simulink model "IEEE33_TR_TEMPORAL_RECOGNIZABILITY_MASTER"  (R2026b)
settings: Solver=ode23t  StopTime=0.2  MaxStep=1e-5
undefined symbols (not defined in the file): Three_PhaseBreaker_class, Three_PhaseSeriesRLCLoad_class, Three_PhaseSource_class, Three_PhaseV_IMeasuremen_class
libraries: ee_lib x146, nesl_utility x106, fl_lib x33, eeRmsMeasurement x2
(part 3 of 7)

== system IEEE33_TR_TEMPORAL_RECOGNIZABILITY_MASTER/Three-Phase Series RLC Branch31 ==
  Three_PhaseSeriesRLCBran : ee_lib/Passive/RLC Assemblies/RLC (Three-Phase)  port_option=ee.enum.threePhasePort.expanded  component_structure=4  R=0.5075 Ohm  L=0.00082283 H  C=1e-06 F  R_parasitic=1e-6 Ohm  G_parasitic=1e-6 1/Ohm  IL_specify=on  IL_priority=High  IL=[0, 0, 0] A  IL_nominal_specify=off  IL_nominal_value=1  IL_nominal_unit=A  VC_specify=on  VC_priority=High  VC=[0, 0, 0] V  VC_nominal_specify=off  VC_nominal_value=1  VC_nominal_unit=V
  A : PMIOPort  Side=Left
  B : PMIOPort  Port=2  Side=Left
  C : PMIOPort  Port=3  Side=Left
  a : PMIOPort  Port=4  Side=Right
  b : PMIOPort  Port=5  Side=Right
  c : PMIOPort  Port=6  Side=Right
  connections:
  Three_PhaseSeriesRLCBran/RConn3 -- c/RConn1
  Three_PhaseSeriesRLCBran/RConn2 -- b/RConn1
  Three_PhaseSeriesRLCBran/RConn1 -- a/RConn1
  C/RConn1 -- Three_PhaseSeriesRLCBran/LConn3
  B/RConn1 -- Three_PhaseSeriesRLCBran/LConn2
  A/RConn1 -- Three_PhaseSeriesRLCBran/LConn1

== system IEEE33_TR_TEMPORAL_RECOGNIZABILITY_MASTER/Three-Phase Series RLC Branch32 ==
  Three_PhaseSeriesRLCBran : ee_lib/Passive/RLC Assemblies/RLC (Three-Phase)  port_option=ee.enum.threePhasePort.expanded  component_structure=4  R=0.9744 Ohm  L=0.0030653 H  C=1e-06 F  R_parasitic=1e-6 Ohm  G_parasitic=1e-6 1/Ohm  IL_specify=on  IL_priority=High  IL=[0, 0, 0] A  IL_nominal_specify=off  IL_nominal_value=1  IL_nominal_unit=A  VC_specify=on  VC_priority=High  VC=[0, 0, 0] V  VC_nominal_specify=off  VC_nominal_value=1  VC_nominal_unit=V
  A : PMIOPort  Side=Left
  B : PMIOPort  Port=2  Side=Left
  C : PMIOPort  Port=3  Side=Left
  a : PMIOPort  Port=4  Side=Right
  b : PMIOPort  Port=5  Side=Right
  c : PMIOPort  Port=6  Side=Right
  connections:
  Three_PhaseSeriesRLCBran/RConn3 -- c/RConn1
  Three_PhaseSeriesRLCBran/RConn2 -- b/RConn1
  Three_PhaseSeriesRLCBran/RConn1 -- a/RConn1
  C/RConn1 -- Three_PhaseSeriesRLCBran/LConn3
  B/RConn1 -- Three_PhaseSeriesRLCBran/LConn2
  A/RConn1 -- Three_PhaseSeriesRLCBran/LConn1

== system IEEE33_TR_TEMPORAL_RECOGNIZABILITY_MASTER/Three-Phase Series RLC Branch33 ==
  Three_PhaseSeriesRLCBran : ee_lib/Passive/RLC Assemblies/RLC (Three-Phase)  port_option=ee.enum.threePhasePort.expanded  component_structure=4  R=0.3105 Ohm  L=0.001152 H  C=1e-06 F  R_parasitic=1e-6 Ohm  G_parasitic=1e-6 1/Ohm  IL_specify=on  IL_priority=High  IL=[0, 0, 0] A  IL_nominal_specify=off  IL_nominal_value=1  IL_nominal_unit=A  VC_specify=on  VC_priority=High  VC=[0, 0, 0] V  VC_nominal_specify=off  VC_nominal_value=1  VC_nominal_unit=V
  A : PMIOPort  Side=Left
  B : PMIOPort  Port=2  Side=Left
  C : PMIOPort  Port=3  Side=Left
  a : PMIOPort  Port=4  Side=Right
  b : PMIOPort  Port=5  Side=Right
  c : PMIOPort  Port=6  Side=Right
  connections:
  Three_PhaseSeriesRLCBran/RConn3 -- c/RConn1
  Three_PhaseSeriesRLCBran/RConn2 -- b/RConn1
  Three_PhaseSeriesRLCBran/RConn1 -- a/RConn1
  C/RConn1 -- Three_PhaseSeriesRLCBran/LConn3
  B/RConn1 -- Three_PhaseSeriesRLCBran/LConn2
  A/RConn1 -- Three_PhaseSeriesRLCBran/LConn1

== system IEEE33_TR_TEMPORAL_RECOGNIZABILITY_MASTER/Three-Phase Series RLC Branch34 ==
  Three_PhaseSeriesRLCBran : ee_lib/Passive/RLC Assemblies/RLC (Three-Phase)  port_option=ee.enum.threePhasePort.expanded  component_structure=4  R=0.341 Ohm  L=0.0016877 H  C=1e-06 F  R_parasitic=1e-6 Ohm  G_parasitic=1e-6 1/Ohm  IL_specify=on  IL_priority=High  IL=[0, 0, 0] A  IL_nominal_specify=off  IL_nominal_value=1  IL_nominal_unit=A  VC_specify=on  VC_priority=High  VC=[0, 0, 0] V  VC_nominal_specify=off  VC_nominal_value=1  VC_nominal_unit=V
  A : PMIOPort  Side=Left
  B : PMIOPort  Port=2  Side=Left
  C : PMIOPort  Port=3  Side=Left
  a : PMIOPort  Port=4  Side=Right
  b : PMIOPort  Port=5  Side=Right
  c : PMIOPort  Port=6  Side=Right
  connections:
  Three_PhaseSeriesRLCBran/RConn3 -- c/RConn1
  Three_PhaseSeriesRLCBran/RConn2 -- b/RConn1
  Three_PhaseSeriesRLCBran/RConn1 -- a/RConn1
  C/RConn1 -- Three_PhaseSeriesRLCBran/LConn3
  B/RConn1 -- Three_PhaseSeriesRLCBran/LConn2
  A/RConn1 -- Three_PhaseSeriesRLCBran/LConn1

== system IEEE33_TR_TEMPORAL_RECOGNIZABILITY_MASTER/Three-Phase Series RLC Branch35 ==
  Three_PhaseSeriesRLCBran : ee_lib/Passive/RLC Assemblies/RLC (Three-Phase)  port_option=ee.enum.threePhasePort.expanded  component_structure=4  R=2 Ohm  L=0.0063662 H  C=1e-06 F  R_parasitic=1e-6 Ohm  G_parasitic=1e-6 1/Ohm  IL_specify=on  IL_priority=High  IL=[0, 0, 0] A  IL_nominal_specify=off  IL_nominal_value=1  IL_nominal_unit=A  VC_specify=on  VC_priority=High  VC=[0, 0, 0] V  VC_nominal_specify=off  VC_nominal_value=1  VC_nominal_unit=V
  A : PMIOPort  Side=Left
  B : PMIOPort  Port=2  Side=Left
  C : PMIOPort  Port=3  Side=Left
  a : PMIOPort  Port=4  Side=Right
  b : PMIOPort  Port=5  Side=Right
  c : PMIOPort  Port=6  Side=Right
  connections:
  Three_PhaseSeriesRLCBran/RConn3 -- c/RConn1
  Three_PhaseSeriesRLCBran/RConn2 -- b/RConn1
  Three_PhaseSeriesRLCBran/RConn1 -- a/RConn1
  C/RConn1 -- Three_PhaseSeriesRLCBran/LConn3
  B/RConn1 -- Three_PhaseSeriesRLCBran/LConn2
  A/RConn1 -- Three_PhaseSeriesRLCBran/LConn1

== system IEEE33_TR_TEMPORAL_RECOGNIZABILITY_MASTER/Three-Phase Series RLC Branch36 ==
  Three_PhaseSeriesRLCBran : ee_lib/Passive/RLC Assemblies/RLC (Three-Phase)  port_option=ee.enum.threePhasePort.expanded  component_structure=4  R=2 Ohm  L=0.0063662 H  C=1e-06 F  R_parasitic=1e-6 Ohm  G_parasitic=1e-6 1/Ohm  IL_specify=on  IL_priority=High  IL=[0, 0, 0] A  IL_nominal_specify=off  IL_nominal_value=1  IL_nominal_unit=A  VC_specify=on  VC_priority=High  VC=[0, 0, 0] V  VC_nominal_specify=off  VC_nominal_value=1  VC_nominal_unit=V
  A : PMIOPort  Side=Left
  B : PMIOPort  Port=2  Side=Left
  C : PMIOPort  Port=3  Side=Left
  a : PMIOPort  Port=4  Side=Right
  b : PMIOPort  Port=5  Side=Right
  c : PMIOPort  Port=6  Side=Right
  connections:
  Three_PhaseSeriesRLCBran/RConn3 -- c/RConn1
  Three_PhaseSeriesRLCBran/RConn2 -- b/RConn1
  Three_PhaseSeriesRLCBran/RConn1 -- a/RConn1
  C/RConn1 -- Three_PhaseSeriesRLCBran/LConn3
  B/RConn1 -- Three_PhaseSeriesRLCBran/LConn2
  A/RConn1 -- Three_PhaseSeriesRLCBran/LConn1

== system IEEE33_TR_TEMPORAL_RECOGNIZABILITY_MASTER/Three-Phase Series RLC Branch37 ==
  Three_PhaseSeriesRLCBran : ee_lib/Passive/RLC Assemblies/RLC (Three-Phase)  port_option=ee.enum.threePhasePort.expanded  component_structure=4  R=0.5 Ohm  L=0.0015915 H  C=1e-06 F  R_parasitic=1e-6 Ohm  G_parasitic=1e-6 1/Ohm  IL_specify=on  IL_priority=High  IL=[0, 0, 0] A  IL_nominal_specify=off  IL_nominal_value=1  IL_nominal_unit=A  VC_specify=on  VC_priority=High  VC=[0, 0, 0] V  VC_nominal_specify=off  VC_nominal_value=1  VC_nominal_unit=V
  A : PMIOPort  Side=Left
  B : PMIOPort  Port=2  Side=Left
  C : PMIOPort  Port=3  Side=Left
  a : PMIOPort  Port=4  Side=Right
  b : PMIOPort  Port=5  Side=Right
  c : PMIOPort  Port=6  Side=Right
  connections:
  Three_PhaseSeriesRLCBran/RConn3 -- c/RConn1
  Three_PhaseSeriesRLCBran/RConn2 -- b/RConn1
  Three_PhaseSeriesRLCBran/RConn1 -- a/RConn1
  C/RConn1 -- Three_PhaseSeriesRLCBran/LConn3
  B/RConn1 -- Three_PhaseSeriesRLCBran/LConn2
  A/RConn1 -- Three_PhaseSeriesRLCBran/LConn1

== system IEEE33_TR_TEMPORAL_RECOGNIZABILITY_MASTER/Three-Phase Series RLC Branch38 ==
  Three_PhaseSeriesRLCBran : ee_lib/Passive/RLC Assemblies/RLC (Three-Phase)  port_option=ee.enum.threePhasePort.expanded  component_structure=4  R=0.5 Ohm  L=0.0015915 H  C=1e-06 F  R_parasitic=1e-6 Ohm  G_parasitic=1e-6 1/Ohm  IL_specify=on  IL_priority=High  IL=[0, 0, 0] A  IL_nominal_specify=off  IL_nominal_value=1  IL_nominal_unit=A  VC_specify=on  VC_priority=High  VC=[0, 0, 0] V  VC_nominal_specify=off  VC_nominal_value=1  VC_nominal_unit=V
  A : PMIOPort  Side=Left
  B : PMIOPort  Port=2  Side=Left
  C : PMIOPort  Port=3  Side=Left
  a : PMIOPort  Port=4  Side=Right
  b : PMIOPort  Port=5  Side=Right
  c : PMIOPort  Port=6  Side=Right
  connections:
  Three_PhaseSeriesRLCBran/RConn3 -- c/RConn1
  Three_PhaseSeriesRLCBran/RConn2 -- b/RConn1
  Three_PhaseSeriesRLCBran/RConn1 -- a/RConn1
  C/RConn1 -- Three_PhaseSeriesRLCBran/LConn3
  B/RConn1 -- Three_PhaseSeriesRLCBran/LConn2
  A/RConn1 -- Three_PhaseSeriesRLCBran/LConn1

== system IEEE33_TR_TEMPORAL_RECOGNIZABILITY_MASTER/Three-Phase Series RLC Branch4 ==
  Three_PhaseSeriesRLCBran : ee_lib/Passive/RLC Assemblies/RLC (Three-Phase)  port_option=ee.enum.threePhasePort.expanded  component_structure=4  R=0.819 Ohm  L=0.0022505 H  C=1e-06 F  R_parasitic=1e-6 Ohm  G_parasitic=1e-6 1/Ohm  IL_specify=on  IL_priority=High  IL=[0, 0, 0] A  IL_nominal_specify=off  IL_nominal_value=1  IL_nominal_unit=A  VC_specify=on  VC_priority=High  VC=[0, 0, 0] V  VC_nominal_specify=off  VC_nominal_value=1  VC_nominal_unit=V
  A : PMIOPort  Side=Left
  B : PMIOPort  Port=2  Side=Left
  C : PMIOPort  Port=3  Side=Left
  a : PMIOPort  Port=4  Side=Right
  b : PMIOPort  Port=5  Side=Right
  c : PMIOPort  Port=6  Side=Right
  connections:
  Three_PhaseSeriesRLCBran/RConn3 -- c/RConn1
  Three_PhaseSeriesRLCBran/RConn2 -- b/RConn1
  Three_PhaseSeriesRLCBran/RConn1 -- a/RConn1
  C/RConn1 -- Three_PhaseSeriesRLCBran/LConn3
  B/RConn1 -- Three_PhaseSeriesRLCBran/LConn2
  A/RConn1 -- Three_PhaseSeriesRLCBran/LConn1

== system IEEE33_TR_TEMPORAL_RECOGNIZABILITY_MASTER/Three-Phase Series RLC Branch5 ==
  Three_PhaseSeriesRLCBran : ee_lib/Passive/RLC Assemblies/RLC (Three-Phase)  port_option=ee.enum.threePhasePort.expanded  component_structure=4  R=0.1872 Ohm  L=0.0019697 H  C=1e-06 F  R_parasitic=1e-6 Ohm  G_parasitic=1e-6 1/Ohm  IL_specify=on  IL_priority=High  IL=[0, 0, 0] A  IL_nominal_specify=off  IL_nominal_value=1  IL_nominal_unit=A  VC_specify=on  VC_priority=High  VC=[0, 0, 0] V  VC_nominal_specify=off  VC_nominal_value=1  VC_nominal_unit=V
  A : PMIOPort  Side=Left
  B : PMIOPort  Port=2  Side=Left
  C : PMIOPort  Port=3  Side=Left
  a : PMIOPort  Port=4  Side=Right
  b : PMIOPort  Port=5  Side=Right
  c : PMIOPort  Port=6  Side=Right
  connections:
  Three_PhaseSeriesRLCBran/RConn3 -- c/RConn1
  Three_PhaseSeriesRLCBran/RConn2 -- b/RConn1
  Three_PhaseSeriesRLCBran/RConn1 -- a/RConn1
  C/RConn1 -- Three_PhaseSeriesRLCBran/LConn3
  B/RConn1 -- Three_PhaseSeriesRLCBran/LConn2
  A/RConn1 -- Three_PhaseSeriesRLCBran/LConn1

== system IEEE33_TR_TEMPORAL_RECOGNIZABILITY_MASTER/Three-Phase Series RLC Branch6 ==
  Three_PhaseSeriesRLCBran : ee_lib/Passive/RLC Assemblies/RLC (Three-Phase)  port_option=ee.enum.threePhasePort.expanded  component_structure=4  R=0.7114 Ohm  L=0.00074835 H  C=1e-06 F  R_parasitic=1e-6 Ohm  G_parasitic=1e-6 1/Ohm  IL_specify=on  IL_priority=High  IL=[0, 0, 0] A  IL_nominal_specify=off  IL_nominal_value=1  IL_nominal_unit=A  VC_specify=on  VC_priority=High  VC=[0, 0, 0] V  VC_nominal_specify=off  VC_nominal_value=1  VC_nominal_unit=V
  A : PMIOPort  Side=Left
  B : PMIOPort  Port=2  Side=Left
  C : PMIOPort  Port=3  Side=Left
  a : PMIOPort  Port=4  Side=Right
  b : PMIOPort  Port=5  Side=Right
  c : PMIOPort  Port=6  Side=Right
  connections:
  Three_PhaseSeriesRLCBran/RConn3 -- c/RConn1
  Three_PhaseSeriesRLCBran/RConn2 -- b/RConn1
  Three_PhaseSeriesRLCBran/RConn1 -- a/RConn1
  C/RConn1 -- Three_PhaseSeriesRLCBran/LConn3
  B/RConn1 -- Three_PhaseSeriesRLCBran/LConn2
  A/RConn1 -- Three_PhaseSeriesRLCBran/LConn1

== system IEEE33_TR_TEMPORAL_RECOGNIZABILITY_MASTER/Three-Phase Series RLC Branch7 ==
  Three_PhaseSeriesRLCBran : ee_lib/Passive/RLC Assemblies/RLC (Three-Phase)  port_option=ee.enum.threePhasePort.expanded  component_structure=4  R=1.03 Ohm  L=0.0023555 H  C=1e-06 F  R_parasitic=1e-6 Ohm  G_parasitic=1e-6 1/Ohm  IL_specify=on  IL_priority=High  IL=[0, 0, 0] A  IL_nominal_specify=off  IL_nominal_value=1  IL_nominal_unit=A  VC_specify=on  VC_priority=High  VC=[0, 0, 0] V  VC_nominal_specify=off  VC_nominal_value=1  VC_nominal_unit=V
  A : PMIOPort  Side=Left
  B : PMIOPort  Port=2  Side=Left
  C : PMIOPort  Port=3  Side=Left
  a : PMIOPort  Port=4  Side=Right
  b : PMIOPort  Port=5  Side=Right
  c : PMIOPort  Port=6  Side=Right
  connections:
  Three_PhaseSeriesRLCBran/RConn3 -- c/RConn1
  Three_PhaseSeriesRLCBran/RConn2 -- b/RConn1
  Three_PhaseSeriesRLCBran/RConn1 -- a/RConn1
  C/RConn1 -- Three_PhaseSeriesRLCBran/LConn3
  B/RConn1 -- Three_PhaseSeriesRLCBran/LConn2
  A/RConn1 -- Three_PhaseSeriesRLCBran/LConn1

== system IEEE33_TR_TEMPORAL_RECOGNIZABILITY_MASTER/Three-Phase Series RLC Branch8 ==
  Three_PhaseSeriesRLCBran : ee_lib/Passive/RLC Assemblies/RLC (Three-Phase)  port_option=ee.enum.threePhasePort.expanded  component_structure=4  R=1.044 Ohm  L=0.0023555 H  C=1e-06 F  R_parasitic=1e-6 Ohm  G_parasitic=1e-6 1/Ohm  IL_specify=on  IL_priority=High  IL=[0, 0, 0] A  IL_nominal_specify=off  IL_nominal_value=1  IL_nominal_unit=A  VC_specify=on  VC_priority=High  VC=[0, 0, 0] V  VC_nominal_specify=off  VC_nominal_value=1  VC_nominal_unit=V
  A : PMIOPort  Side=Left
  B : PMIOPort  Port=2  Side=Left
  C : PMIOPort  Port=3  Side=Left
  a : PMIOPort  Port=4  Side=Right
  b : PMIOPort  Port=5  Side=Right
  c : PMIOPort  Port=6  Side=Right
  connections:
  Three_PhaseSeriesRLCBran/RConn3 -- c/RConn1
  Three_PhaseSeriesRLCBran/RConn2 -- b/RConn1
  Three_PhaseSeriesRLCBran/RConn1 -- a/RConn1
  C/RConn1 -- Three_PhaseSeriesRLCBran/LConn3
  B/RConn1 -- Three_PhaseSeriesRLCBran/LConn2
  A/RConn1 -- Three_PhaseSeriesRLCBran/LConn1

== system IEEE33_TR_TEMPORAL_RECOGNIZABILITY_MASTER/Three-Phase Series RLC Branch9 ==
  Three_PhaseSeriesRLCBran : ee_lib/Passive/RLC Assemblies/RLC (Three-Phase)  port_option=ee.enum.threePhasePort.expanded  component_structure=4  R=0.1966 Ohm  L=0.0002069 H  C=1e-06 F  R_parasitic=1e-6 Ohm  G_parasitic=1e-6 1/Ohm  IL_specify=on  IL_priority=High  IL=[0, 0, 0] A  IL_nominal_specify=off  IL_nominal_value=1  IL_nominal_unit=A  VC_specify=on  VC_priority=High  VC=[0, 0, 0] V  VC_nominal_specify=off  VC_nominal_value=1  VC_nominal_unit=V
  A : PMIOPort  Side=Left
  B : PMIOPort  Port=2  Side=Left
  C : PMIOPort  Port=3  Side=Left
  a : PMIOPort  Port=4  Side=Right
  b : PMIOPort  Port=5  Side=Right
  c : PMIOPort  Port=6  Side=Right
  connections:
  Three_PhaseSeriesRLCBran/RConn3 -- c/RConn1
  Three_PhaseSeriesRLCBran/RConn2 -- b/RConn1
  Three_PhaseSeriesRLCBran/RConn1 -- a/RConn1
  C/RConn1 -- Three_PhaseSeriesRLCBran/LConn3
  B/RConn1 -- Three_PhaseSeriesRLCBran/LConn2
  A/RConn1 -- Three_PhaseSeriesRLCBran/LConn1

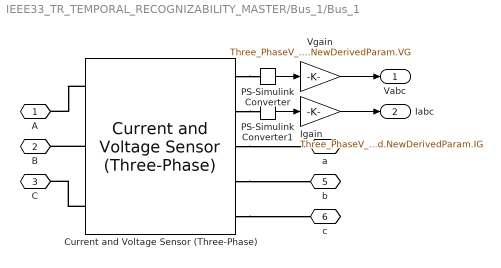
== system IEEE33_TR_TEMPORAL_RECOGNIZABILITY_MASTER/Bus_1/Bus_1 ==
  Current and Voltage Sensor (Three-Phase) : ee_lib/Sensors & Transducers/Current and Voltage Sensor (Three-Phase)  port_option=ee.enum.threePhasePort.expanded  vMeasurementType=1  outputUnit=2  SRated=100000000 V*A  VRated=500000 V  I_specify=off  I_priority=None  I=[ 0 0 0 ] A  I_nominal_specify=off  I_nominal_value=1  I_nominal_unit=A  V_specify=off  V_priority=None  V=[ 0 0 0 ] V  V_nominal_specify=off  V_nominal_value=1  V_nominal_unit=V
  Igain : Gain  Gain=Three_PhaseV_IMeasuremen_class('phase-to-phase','yes','off','off','off',100000000,500000).objParamMappingDerived.NewDerivedParam.IG
  PS-Simulink Converter : nesl_utility/PS-Simulink Converter  PhysicalDomain=network_engine_domain  SubClassName=ps_output  LeftPortType=input  RightPortType=output  PseudoPeriodic=off  Frequencies=[]  VectorFormat=1-D array  Unit=1  AffineConversion=off
  PS-Simulink Converter1 : nesl_utility/PS-Simulink Converter  PhysicalDomain=network_engine_domain  SubClassName=ps_output  LeftPortType=input  RightPortType=output  PseudoPeriodic=off  Frequencies=[]  VectorFormat=1-D array  Unit=1  AffineConversion=off
  Vgain : Gain  Gain=Three_PhaseV_IMeasuremen_class('phase-to-phase','yes','off','off','off',100000000,500000).objParamMappingDerived.NewDerivedParam.VG
  A : PMIOPort  Side=Left
  B : PMIOPort  Port=2  Side=Left
  C : PMIOPort  Port=3  Side=Left
  a : PMIOPort  Port=4  Side=Right
  b : PMIOPort  Port=5  Side=Right
  c : PMIOPort  Port=6  Side=Right
  Vabc : Outport  VectorParamsAs1DForOutWhenUnconnected=off
  Iabc : Outport  Port=2  VectorParamsAs1DForOutWhenUnconnected=off
  wires:
  Igain/1 -> Iabc/1
  Vgain/1 -> Vabc/1
  PS-Simulink Converter1/1 -> Igain/1
  PS-Simulink Converter/1 -> Vgain/1
  connections:
  Current and Voltage Sensor (Three-Phase)/RConn1 -- PS-Simulink Converter/LConn1
  Current and Voltage Sensor (Three-Phase)/RConn2 -- PS-Simulink Converter1/LConn1
  Current and Voltage Sensor (Three-Phase)/RConn5 -- c/RConn1
  Current and Voltage Sensor (Three-Phase)/RConn4 -- b/RConn1
  Current and Voltage Sensor (Three-Phase)/RConn3 -- a/RConn1
  Current and Voltage Sensor (Three-Phase)/LConn3 -- C/RConn1
  Current and Voltage Sensor (Three-Phase)/LConn1 -- A/RConn1
  Current and Voltage Sensor (Three-Phase)/LConn2 -- B/RConn1

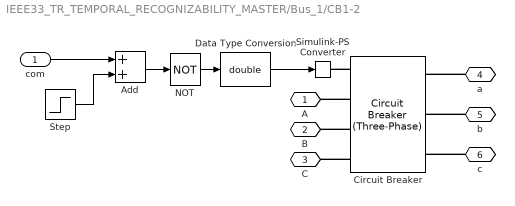
== system IEEE33_TR_TEMPORAL_RECOGNIZABILITY_MASTER/Bus_1/CB1-2 ==
  com : Inport
  Add : Sum
  Circuit Breaker : ee_lib/Switches & Breakers/Circuit Breaker (Three-Phase)  port_option=ee.enum.threePhasePort.expanded  control_port_option=ee.enum.controlport.ps  R_closed=0.01 Ohm  G_open=Three_PhaseBreaker_class('open',1000000,Inf,[0.0166666666666667 0.0833333333333333],'on').objParamMappingDerived.NewDerivedParam.G_open 1/Ohm  threshold=0.5 V  breaker_behavior=ee.enum.switches.breakerBehavior.zeroCrossingEnable  i_th=1e-8 A
  Data Type Conversion : DataTypeConversion  OutDataTypeStr=double  SaturateOnIntegerOverflow=off  RndMeth=Floor
  NOT : Logic  Operator=NOT  IconShape=distinctive  AllPortsSameDT=off  OutDataTypeStr=boolean
  Simulink-PS Converter : nesl_utility/Simulink-PS Converter  PhysicalDomain=network_engine_domain  SubClassName=ps_input  LeftPortType=input  RightPortType=output  PseudoPeriodic=off  Frequencies=[]  NoiseDistribution=none  NoiseParameters=[]  Unit=1  AffineConversion=off  FilteringAndDerivatives=provide  SimscapeFilterOrder=1  InputFilterTimeConstant=0.001  UdotUserProvided=0
  Step : Step  Time=1e-6  InitialValue=Three_PhaseBreaker_class('open',1000000,Inf,[0.0166666666666667 0.0833333333333333],'on').objParamMappingDerived.NewDerivedParam.StepInitialValue  FinalValue=0  SampleTime=0
  A : PMIOPort  Side=Left
  B : PMIOPort  Port=2  Side=Left
  C : PMIOPort  Port=3  Side=Left
  a : PMIOPort  Port=4  Side=Right
  b : PMIOPort  Port=5  Side=Right
  c : PMIOPort  Port=6  Side=Right
  wires:
  com/1 -> Add/1
  Add/1 -> NOT/1
  Step/1 -> Add/2
  Data Type Conversion/1 -> Simulink-PS Converter/1
  NOT/1 -> Data Type Conversion/1
  connections:
  Circuit Breaker/LConn1 -- Simulink-PS Converter/RConn1
  c/RConn1 -- Circuit Breaker/RConn3
  b/RConn1 -- Circuit Breaker/RConn2
  a/RConn1 -- Circuit Breaker/RConn1
  Circuit Breaker/LConn4 -- C/RConn1
  Circuit Breaker/LConn3 -- B/RConn1
  Circuit Breaker/LConn2 -- A/RConn1

== system IEEE33_TR_TEMPORAL_RECOGNIZABILITY_MASTER/Bus_10/Bus Load 10 ==
  Electrical Reference : fl_lib/Electrical/Electrical Elements/Electrical Reference
  Wye-Connected Load : ee_lib/Passive/RLC Assemblies/Wye-Connected Load  port_option=ee.enum.threePhasePort.expanded  parameterization=2  component_structure=4  component_structure_PQ=4  R=1 Ohm  L=0.001 H  C=1e-6 F  VRated=11765.4824 V  FRated=60 Hz  P=60000 W  Qpos=20000 V*A  Qneg=Three_PhaseSeriesRLCLoad_class(0).objParamMappingDerived.NewDerivedParam.Qneg V*A  R_parasitic=1e-6 Ohm  G_parasitic=1e-6 1/Ohm  R_parasitic_PQ=1e-6 Ohm  G_parasitic_PQ=1e-6 1/Ohm  Vmag0=11765.4824 V  Vang0=0 deg  Freq0=60 Hz  IL_specify=on  IL_priority=High  IL=[ 0 0 0 ] A  IL_nominal_specify=off  IL_nominal_value=1  IL_nominal_unit=A  VC_specify=on  VC_priority=High  VC=[ 0 0 0 ] V  VC_nominal_specify=off  VC_nominal_value=1  VC_nominal_unit=V
  A : PMIOPort  Side=Left
  B : PMIOPort  Port=2  Side=Left
  C : PMIOPort  Port=3  Side=Left
  connections:
  Electrical Reference/LConn1 -- Wye-Connected Load/RConn1
  Wye-Connected Load/LConn3 -- C/RConn1
  Wye-Connected Load/LConn1 -- A/RConn1
  Wye-Connected Load/LConn2 -- B/RConn1

== system IEEE33_TR_TEMPORAL_RECOGNIZABILITY_MASTER/Bus_10/Bus_10 ==
  Current and Voltage Sensor (Three-Phase) : ee_lib/Sensors & Transducers/Current and Voltage Sensor (Three-Phase)  port_option=ee.enum.threePhasePort.expanded  vMeasurementType=1  outputUnit=2  SRated=100000000 V*A  VRated=500000 V  I_specify=off  I_priority=None  I=[ 0 0 0 ] A  I_nominal_specify=off  I_nominal_value=1  I_nominal_unit=A  V_specify=off  V_priority=None  V=[ 0 0 0 ] V  V_nominal_specify=off  V_nominal_value=1  V_nominal_unit=V
  Igain : Gain  Gain=Three_PhaseV_IMeasuremen_class('phase-to-phase','yes','off','off','off',100000000,500000).objParamMappingDerived.NewDerivedParam.IG
  PS-Simulink Converter : nesl_utility/PS-Simulink Converter  PhysicalDomain=network_engine_domain  SubClassName=ps_output  LeftPortType=input  RightPortType=output  PseudoPeriodic=off  Frequencies=[]  VectorFormat=1-D array  Unit=1  AffineConversion=off
  PS-Simulink Converter1 : nesl_utility/PS-Simulink Converter  PhysicalDomain=network_engine_domain  SubClassName=ps_output  LeftPortType=input  RightPortType=output  PseudoPeriodic=off  Frequencies=[]  VectorFormat=1-D array  Unit=1  AffineConversion=off
  Vgain : Gain  Gain=Three_PhaseV_IMeasuremen_class('phase-to-phase','yes','off','off','off',100000000,500000).objParamMappingDerived.NewDerivedParam.VG
  A : PMIOPort  Side=Left
  B : PMIOPort  Port=2  Side=Left
  C : PMIOPort  Port=3  Side=Left
  a : PMIOPort  Port=4  Side=Right
  b : PMIOPort  Port=5  Side=Right
  c : PMIOPort  Port=6  Side=Right
  Vabc : Outport  VectorParamsAs1DForOutWhenUnconnected=off
  Iabc : Outport  Port=2  VectorParamsAs1DForOutWhenUnconnected=off
  wires:
  Igain/1 -> Iabc/1
  Vgain/1 -> Vabc/1
  PS-Simulink Converter1/1 -> Igain/1
  PS-Simulink Converter/1 -> Vgain/1
  connections:
  Current and Voltage Sensor (Three-Phase)/RConn1 -- PS-Simulink Converter/LConn1
  Current and Voltage Sensor (Three-Phase)/RConn2 -- PS-Simulink Converter1/LConn1
  Current and Voltage Sensor (Three-Phase)/RConn5 -- c/RConn1
  Current and Voltage Sensor (Three-Phase)/RConn4 -- b/RConn1
  Current and Voltage Sensor (Three-Phase)/RConn3 -- a/RConn1
  Current and Voltage Sensor (Three-Phase)/LConn3 -- C/RConn1
  Current and Voltage Sensor (Three-Phase)/LConn1 -- A/RConn1
  Current and Voltage Sensor (Three-Phase)/LConn2 -- B/RConn1

== system IEEE33_TR_TEMPORAL_RECOGNIZABILITY_MASTER/Bus_10/CB3-2 ==
  com : Inport
  Add : Sum
  Circuit Breaker : ee_lib/Switches & Breakers/Circuit Breaker (Three-Phase)  port_option=ee.enum.threePhasePort.expanded  control_port_option=ee.enum.controlport.ps  R_closed=0.01 Ohm  G_open=Three_PhaseBreaker_class('open',1000000,Inf,[0.0166666666666667 0.0833333333333333],'on').objParamMappingDerived.NewDerivedParam.G_open 1/Ohm  threshold=0.5 V  breaker_behavior=ee.enum.switches.breakerBehavior.zeroCrossingEnable  i_th=1e-8 A
  Data Type Conversion : DataTypeConversion  OutDataTypeStr=double  SaturateOnIntegerOverflow=off  RndMeth=Floor
  NOT : Logic  Operator=NOT  IconShape=distinctive  AllPortsSameDT=off  OutDataTypeStr=boolean
  Simulink-PS Converter : nesl_utility/Simulink-PS Converter  PhysicalDomain=network_engine_domain  SubClassName=ps_input  LeftPortType=input  RightPortType=output  PseudoPeriodic=off  Frequencies=[]  NoiseDistribution=none  NoiseParameters=[]  Unit=1  AffineConversion=off  FilteringAndDerivatives=provide  SimscapeFilterOrder=1  InputFilterTimeConstant=0.001  UdotUserProvided=0
  Step : Step  Time=1e-6  InitialValue=Three_PhaseBreaker_class('open',1000000,Inf,[0.0166666666666667 0.0833333333333333],'on').objParamMappingDerived.NewDerivedParam.StepInitialValue  FinalValue=0  SampleTime=0
  A : PMIOPort  Side=Left
  B : PMIOPort  Port=2  Side=Left
  C : PMIOPort  Port=3  Side=Left
  a : PMIOPort  Port=4  Side=Right
  b : PMIOPort  Port=5  Side=Right
  c : PMIOPort  Port=6  Side=Right
  wires:
  com/1 -> Add/1
  Add/1 -> NOT/1
  Step/1 -> Add/2
  Data Type Conversion/1 -> Simulink-PS Converter/1
  NOT/1 -> Data Type Conversion/1
  connections:
  Circuit Breaker/LConn1 -- Simulink-PS Converter/RConn1
  c/RConn1 -- Circuit Breaker/RConn3
  b/RConn1 -- Circuit Breaker/RConn2
  a/RConn1 -- Circuit Breaker/RConn1
  Circuit Breaker/LConn4 -- C/RConn1
  Circuit Breaker/LConn3 -- B/RConn1
  Circuit Breaker/LConn2 -- A/RConn1

== system IEEE33_TR_TEMPORAL_RECOGNIZABILITY_MASTER/Bus_10/VI Recorder13 ==
  Vrec : Inport
  Irec : Inport  Port=2
  tag scope: I9to10=global, V9to10=global
  wires:
  Vrec/1 -> [V9to10]
  Irec/1 -> [I9to10]

== system IEEE33_TR_TEMPORAL_RECOGNIZABILITY_MASTER/Bus_11/Bus Load 11 ==
  Electrical Reference : fl_lib/Electrical/Electrical Elements/Electrical Reference
  Wye-Connected Load : ee_lib/Passive/RLC Assemblies/Wye-Connected Load  port_option=ee.enum.threePhasePort.expanded  parameterization=2  component_structure=4  component_structure_PQ=4  R=1 Ohm  L=0.001 H  C=1e-6 F  VRated=11754.6201 V  FRated=60 Hz  P=45000 W  Qpos=30000 V*A  Qneg=Three_PhaseSeriesRLCLoad_class(0).objParamMappingDerived.NewDerivedParam.Qneg V*A  R_parasitic=1e-6 Ohm  G_parasitic=1e-6 1/Ohm  R_parasitic_PQ=1e-6 Ohm  G_parasitic_PQ=1e-6 1/Ohm  Vmag0=11754.6201 V  Vang0=0 deg  Freq0=60 Hz  IL_specify=on  IL_priority=High  IL=[ 0 0 0 ] A  IL_nominal_specify=off  IL_nominal_value=1  IL_nominal_unit=A  VC_specify=on  VC_priority=High  VC=[ 0 0 0 ] V  VC_nominal_specify=off  VC_nominal_value=1  VC_nominal_unit=V
  A : PMIOPort  Side=Left
  B : PMIOPort  Port=2  Side=Left
  C : PMIOPort  Port=3  Side=Left
  connections:
  Electrical Reference/LConn1 -- Wye-Connected Load/RConn1
  Wye-Connected Load/LConn3 -- C/RConn1
  Wye-Connected Load/LConn1 -- A/RConn1
  Wye-Connected Load/LConn2 -- B/RConn1

== system IEEE33_TR_TEMPORAL_RECOGNIZABILITY_MASTER/Bus_11/Bus_11 ==
  Current and Voltage Sensor (Three-Phase) : ee_lib/Sensors & Transducers/Current and Voltage Sensor (Three-Phase)  port_option=ee.enum.threePhasePort.expanded  vMeasurementType=1  outputUnit=2  SRated=100000000 V*A  VRated=500000 V  I_specify=off  I_priority=None  I=[ 0 0 0 ] A  I_nominal_specify=off  I_nominal_value=1  I_nominal_unit=A  V_specify=off  V_priority=None  V=[ 0 0 0 ] V  V_nominal_specify=off  V_nominal_value=1  V_nominal_unit=V
  Igain : Gain  Gain=Three_PhaseV_IMeasuremen_class('phase-to-phase','yes','off','off','off',100000000,500000).objParamMappingDerived.NewDerivedParam.IG
  PS-Simulink Converter : nesl_utility/PS-Simulink Converter  PhysicalDomain=network_engine_domain  SubClassName=ps_output  LeftPortType=input  RightPortType=output  PseudoPeriodic=off  Frequencies=[]  VectorFormat=1-D array  Unit=1  AffineConversion=off
  PS-Simulink Converter1 : nesl_utility/PS-Simulink Converter  PhysicalDomain=network_engine_domain  SubClassName=ps_output  LeftPortType=input  RightPortType=output  PseudoPeriodic=off  Frequencies=[]  VectorFormat=1-D array  Unit=1  AffineConversion=off
  Vgain : Gain  Gain=Three_PhaseV_IMeasuremen_class('phase-to-phase','yes','off','off','off',100000000,500000).objParamMappingDerived.NewDerivedParam.VG
  A : PMIOPort  Side=Left
  B : PMIOPort  Port=2  Side=Left
  C : PMIOPort  Port=3  Side=Left
  a : PMIOPort  Port=4  Side=Right
  b : PMIOPort  Port=5  Side=Right
  c : PMIOPort  Port=6  Side=Right
  Vabc : Outport  VectorParamsAs1DForOutWhenUnconnected=off
  Iabc : Outport  Port=2  VectorParamsAs1DForOutWhenUnconnected=off
  wires:
  Igain/1 -> Iabc/1
  Vgain/1 -> Vabc/1
  PS-Simulink Converter1/1 -> Igain/1
  PS-Simulink Converter/1 -> Vgain/1
  connections:
  Current and Voltage Sensor (Three-Phase)/RConn1 -- PS-Simulink Converter/LConn1
  Current and Voltage Sensor (Three-Phase)/RConn2 -- PS-Simulink Converter1/LConn1
  Current and Voltage Sensor (Three-Phase)/RConn5 -- c/RConn1
  Current and Voltage Sensor (Three-Phase)/RConn4 -- b/RConn1
  Current and Voltage Sensor (Three-Phase)/RConn3 -- a/RConn1
  Current and Voltage Sensor (Three-Phase)/LConn3 -- C/RConn1
  Current and Voltage Sensor (Three-Phase)/LConn1 -- A/RConn1
  Current and Voltage Sensor (Three-Phase)/LConn2 -- B/RConn1

== system IEEE33_TR_TEMPORAL_RECOGNIZABILITY_MASTER/Bus_11/CB3-2 ==
  com : Inport
  Add : Sum
  Circuit Breaker : ee_lib/Switches & Breakers/Circuit Breaker (Three-Phase)  port_option=ee.enum.threePhasePort.expanded  control_port_option=ee.enum.controlport.ps  R_closed=0.01 Ohm  G_open=Three_PhaseBreaker_class('open',1000000,Inf,[0.0166666666666667 0.0833333333333333],'on').objParamMappingDerived.NewDerivedParam.G_open 1/Ohm  threshold=0.5 V  breaker_behavior=ee.enum.switches.breakerBehavior.zeroCrossingEnable  i_th=1e-8 A
  Data Type Conversion : DataTypeConversion  OutDataTypeStr=double  SaturateOnIntegerOverflow=off  RndMeth=Floor
  NOT : Logic  Operator=NOT  IconShape=distinctive  AllPortsSameDT=off  OutDataTypeStr=boolean
  Simulink-PS Converter : nesl_utility/Simulink-PS Converter  PhysicalDomain=network_engine_domain  SubClassName=ps_input  LeftPortType=input  RightPortType=output  PseudoPeriodic=off  Frequencies=[]  NoiseDistribution=none  NoiseParameters=[]  Unit=1  AffineConversion=off  FilteringAndDerivatives=provide  SimscapeFilterOrder=1  InputFilterTimeConstant=0.001  UdotUserProvided=0
  Step : Step  Time=1e-6  InitialValue=Three_PhaseBreaker_class('open',1000000,Inf,[0.0166666666666667 0.0833333333333333],'on').objParamMappingDerived.NewDerivedParam.StepInitialValue  FinalValue=0  SampleTime=0
  A : PMIOPort  Side=Left
  B : PMIOPort  Port=2  Side=Left
  C : PMIOPort  Port=3  Side=Left
  a : PMIOPort  Port=4  Side=Right
  b : PMIOPort  Port=5  Side=Right
  c : PMIOPort  Port=6  Side=Right
  wires:
  com/1 -> Add/1
  Add/1 -> NOT/1
  Step/1 -> Add/2
  Data Type Conversion/1 -> Simulink-PS Converter/1
  NOT/1 -> Data Type Conversion/1
  connections:
  Circuit Breaker/LConn1 -- Simulink-PS Converter/RConn1
  c/RConn1 -- Circuit Breaker/RConn3
  b/RConn1 -- Circuit Breaker/RConn2
  a/RConn1 -- Circuit Breaker/RConn1
  Circuit Breaker/LConn4 -- C/RConn1
  Circuit Breaker/LConn3 -- B/RConn1
  Circuit Breaker/LConn2 -- A/RConn1

== system IEEE33_TR_TEMPORAL_RECOGNIZABILITY_MASTER/Bus_11/VI Recorder14 ==
  Vrec : Inport
  Irec : Inport  Port=2
  tag scope: I10to11=global, V10to11=global
  wires:
  Vrec/1 -> [V10to11]
  Irec/1 -> [I10to11]

== system IEEE33_TR_TEMPORAL_RECOGNIZABILITY_MASTER/Bus_12/Bus Load 12 ==
  Electrical Reference : fl_lib/Electrical/Electrical Elements/Electrical Reference
  Wye-Connected Load : ee_lib/Passive/RLC Assemblies/Wye-Connected Load  port_option=ee.enum.threePhasePort.expanded  parameterization=2  component_structure=4  component_structure_PQ=4  R=1 Ohm  L=0.001 H  C=1e-6 F  VRated=11735.6681 V  FRated=60 Hz  P=60000 W  Qpos=35000 V*A  Qneg=Three_PhaseSeriesRLCLoad_class(0).objParamMappingDerived.NewDerivedParam.Qneg V*A  R_parasitic=1e-6 Ohm  G_parasitic=1e-6 1/Ohm  R_parasitic_PQ=1e-6 Ohm  G_parasitic_PQ=1e-6 1/Ohm  Vmag0=11735.6681 V  Vang0=0 deg  Freq0=60 Hz  IL_specify=on  IL_priority=High  IL=[ 0 0 0 ] A  IL_nominal_specify=off  IL_nominal_value=1  IL_nominal_unit=A  VC_specify=on  VC_priority=High  VC=[ 0 0 0 ] V  VC_nominal_specify=off  VC_nominal_value=1  VC_nominal_unit=V
  A : PMIOPort  Side=Left
  B : PMIOPort  Port=2  Side=Left
  C : PMIOPort  Port=3  Side=Left
  connections:
  Electrical Reference/LConn1 -- Wye-Connected Load/RConn1
  Wye-Connected Load/LConn3 -- C/RConn1
  Wye-Connected Load/LConn1 -- A/RConn1
  Wye-Connected Load/LConn2 -- B/RConn1

== system IEEE33_TR_TEMPORAL_RECOGNIZABILITY_MASTER/Bus_12/Bus_12 ==
  Current and Voltage Sensor (Three-Phase) : ee_lib/Sensors & Transducers/Current and Voltage Sensor (Three-Phase)  port_option=ee.enum.threePhasePort.expanded  vMeasurementType=1  outputUnit=2  SRated=100000000 V*A  VRated=500000 V  I_specify=off  I_priority=None  I=[ 0 0 0 ] A  I_nominal_specify=off  I_nominal_value=1  I_nominal_unit=A  V_specify=off  V_priority=None  V=[ 0 0 0 ] V  V_nominal_specify=off  V_nominal_value=1  V_nominal_unit=V
  Igain : Gain  Gain=Three_PhaseV_IMeasuremen_class('phase-to-phase','yes','off','off','off',100000000,500000).objParamMappingDerived.NewDerivedParam.IG
  PS-Simulink Converter : nesl_utility/PS-Simulink Converter  PhysicalDomain=network_engine_domain  SubClassName=ps_output  LeftPortType=input  RightPortType=output  PseudoPeriodic=off  Frequencies=[]  VectorFormat=1-D array  Unit=1  AffineConversion=off
  PS-Simulink Converter1 : nesl_utility/PS-Simulink Converter  PhysicalDomain=network_engine_domain  SubClassName=ps_output  LeftPortType=input  RightPortType=output  PseudoPeriodic=off  Frequencies=[]  VectorFormat=1-D array  Unit=1  AffineConversion=off
  Vgain : Gain  Gain=Three_PhaseV_IMeasuremen_class('phase-to-phase','yes','off','off','off',100000000,500000).objParamMappingDerived.NewDerivedParam.VG
  A : PMIOPort  Side=Left
  B : PMIOPort  Port=2  Side=Left
  C : PMIOPort  Port=3  Side=Left
  a : PMIOPort  Port=4  Side=Right
  b : PMIOPort  Port=5  Side=Right
  c : PMIOPort  Port=6  Side=Right
  Vabc : Outport  VectorParamsAs1DForOutWhenUnconnected=off
  Iabc : Outport  Port=2  VectorParamsAs1DForOutWhenUnconnected=off
  wires:
  Igain/1 -> Iabc/1
  Vgain/1 -> Vabc/1
  PS-Simulink Converter1/1 -> Igain/1
  PS-Simulink Converter/1 -> Vgain/1
  connections:
  Current and Voltage Sensor (Three-Phase)/RConn1 -- PS-Simulink Converter/LConn1
  Current and Voltage Sensor (Three-Phase)/RConn2 -- PS-Simulink Converter1/LConn1
  Current and Voltage Sensor (Three-Phase)/RConn5 -- c/RConn1
  Current and Voltage Sensor (Three-Phase)/RConn4 -- b/RConn1
  Current and Voltage Sensor (Three-Phase)/RConn3 -- a/RConn1
  Current and Voltage Sensor (Three-Phase)/LConn3 -- C/RConn1
  Current and Voltage Sensor (Three-Phase)/LConn1 -- A/RConn1
  Current and Voltage Sensor (Three-Phase)/LConn2 -- B/RConn1

== system IEEE33_TR_TEMPORAL_RECOGNIZABILITY_MASTER/Bus_12/CB3-2 ==
  com : Inport
  Add : Sum
  Circuit Breaker : ee_lib/Switches & Breakers/Circuit Breaker (Three-Phase)  port_option=ee.enum.threePhasePort.expanded  control_port_option=ee.enum.controlport.ps  R_closed=0.01 Ohm  G_open=Three_PhaseBreaker_class('open',1000000,Inf,[0.0166666666666667 0.0833333333333333],'on').objParamMappingDerived.NewDerivedParam.G_open 1/Ohm  threshold=0.5 V  breaker_behavior=ee.enum.switches.breakerBehavior.zeroCrossingEnable  i_th=1e-8 A
  Data Type Conversion : DataTypeConversion  OutDataTypeStr=double  SaturateOnIntegerOverflow=off  RndMeth=Floor
  NOT : Logic  Operator=NOT  IconShape=distinctive  AllPortsSameDT=off  OutDataTypeStr=boolean
  Simulink-PS Converter : nesl_utility/Simulink-PS Converter  PhysicalDomain=network_engine_domain  SubClassName=ps_input  LeftPortType=input  RightPortType=output  PseudoPeriodic=off  Frequencies=[]  NoiseDistribution=none  NoiseParameters=[]  Unit=1  AffineConversion=off  FilteringAndDerivatives=provide  SimscapeFilterOrder=1  InputFilterTimeConstant=0.001  UdotUserProvided=0
  Step : Step  Time=1e-6  InitialValue=Three_PhaseBreaker_class('open',1000000,Inf,[0.0166666666666667 0.0833333333333333],'on').objParamMappingDerived.NewDerivedParam.StepInitialValue  FinalValue=0  SampleTime=0
  A : PMIOPort  Side=Left
  B : PMIOPort  Port=2  Side=Left
  C : PMIOPort  Port=3  Side=Left
  a : PMIOPort  Port=4  Side=Right
  b : PMIOPort  Port=5  Side=Right
  c : PMIOPort  Port=6  Side=Right
  wires:
  com/1 -> Add/1
  Add/1 -> NOT/1
  Step/1 -> Add/2
  Data Type Conversion/1 -> Simulink-PS Converter/1
  NOT/1 -> Data Type Conversion/1
  connections:
  Circuit Breaker/LConn1 -- Simulink-PS Converter/RConn1
  c/RConn1 -- Circuit Breaker/RConn3
  b/RConn1 -- Circuit Breaker/RConn2
  a/RConn1 -- Circuit Breaker/RConn1
  Circuit Breaker/LConn4 -- C/RConn1
  Circuit Breaker/LConn3 -- B/RConn1
  Circuit Breaker/LConn2 -- A/RConn1

== system IEEE33_TR_TEMPORAL_RECOGNIZABILITY_MASTER/Bus_12/VI Recorder15 ==
  Vrec : Inport
  Irec : Inport  Port=2
  tag scope: I11to12=global, V11to12=global
  wires:
  Vrec/1 -> [V11to12]
  Irec/1 -> [I11to12]

== system IEEE33_TR_TEMPORAL_RECOGNIZABILITY_MASTER/Bus_13/Bus Load 13 ==
  Electrical Reference : fl_lib/Electrical/Electrical Elements/Electrical Reference
  Wye-Connected Load : ee_lib/Passive/RLC Assemblies/Wye-Connected Load  port_option=ee.enum.threePhasePort.expanded  parameterization=2  component_structure=4  component_structure_PQ=4  R=1 Ohm  L=0.001 H  C=1e-6 F  VRated=11658.4168 V  FRated=60 Hz  P=60000 W  Qpos=35000 V*A  Qneg=Three_PhaseSeriesRLCLoad_class(0).objParamMappingDerived.NewDerivedParam.Qneg V*A  R_parasitic=1e-6 Ohm  G_parasitic=1e-6 1/Ohm  R_parasitic_PQ=1e-6 Ohm  G_parasitic_PQ=1e-6 1/Ohm  Vmag0=11658.4168 V  Vang0=0 deg  Freq0=60 Hz  IL_specify=on  IL_priority=High  IL=[ 0 0 0 ] A  IL_nominal_specify=off  IL_nominal_value=1  IL_nominal_unit=A  VC_specify=on  VC_priority=High  VC=[ 0 0 0 ] V  VC_nominal_specify=off  VC_nominal_value=1  VC_nominal_unit=V
  A : PMIOPort  Side=Left
  B : PMIOPort  Port=2  Side=Left
  C : PMIOPort  Port=3  Side=Left
  connections:
  Electrical Reference/LConn1 -- Wye-Connected Load/RConn1
  Wye-Connected Load/LConn3 -- C/RConn1
  Wye-Connected Load/LConn1 -- A/RConn1
  Wye-Connected Load/LConn2 -- B/RConn1

== system IEEE33_TR_TEMPORAL_RECOGNIZABILITY_MASTER/Bus_13/Bus_13 ==
  Current and Voltage Sensor (Three-Phase) : ee_lib/Sensors & Transducers/Current and Voltage Sensor (Three-Phase)  port_option=ee.enum.threePhasePort.expanded  vMeasurementType=1  outputUnit=2  SRated=100000000 V*A  VRated=500000 V  I_specify=off  I_priority=None  I=[ 0 0 0 ] A  I_nominal_specify=off  I_nominal_value=1  I_nominal_unit=A  V_specify=off  V_priority=None  V=[ 0 0 0 ] V  V_nominal_specify=off  V_nominal_value=1  V_nominal_unit=V
  Igain : Gain  Gain=Three_PhaseV_IMeasuremen_class('phase-to-phase','yes','off','off','off',100000000,500000).objParamMappingDerived.NewDerivedParam.IG
  PS-Simulink Converter : nesl_utility/PS-Simulink Converter  PhysicalDomain=network_engine_domain  SubClassName=ps_output  LeftPortType=input  RightPortType=output  PseudoPeriodic=off  Frequencies=[]  VectorFormat=1-D array  Unit=1  AffineConversion=off
  PS-Simulink Converter1 : nesl_utility/PS-Simulink Converter  PhysicalDomain=network_engine_domain  SubClassName=ps_output  LeftPortType=input  RightPortType=output  PseudoPeriodic=off  Frequencies=[]  VectorFormat=1-D array  Unit=1  AffineConversion=off
  Vgain : Gain  Gain=Three_PhaseV_IMeasuremen_class('phase-to-phase','yes','off','off','off',100000000,500000).objParamMappingDerived.NewDerivedParam.VG
  A : PMIOPort  Side=Left
  B : PMIOPort  Port=2  Side=Left
  C : PMIOPort  Port=3  Side=Left
  a : PMIOPort  Port=4  Side=Right
  b : PMIOPort  Port=5  Side=Right
  c : PMIOPort  Port=6  Side=Right
  Vabc : Outport  VectorParamsAs1DForOutWhenUnconnected=off
  Iabc : Outport  Port=2  VectorParamsAs1DForOutWhenUnconnected=off
  wires:
  Igain/1 -> Iabc/1
  Vgain/1 -> Vabc/1
  PS-Simulink Converter1/1 -> Igain/1
  PS-Simulink Converter/1 -> Vgain/1
  connections:
  Current and Voltage Sensor (Three-Phase)/RConn1 -- PS-Simulink Converter/LConn1
  Current and Voltage Sensor (Three-Phase)/RConn2 -- PS-Simulink Converter1/LConn1
  Current and Voltage Sensor (Three-Phase)/RConn5 -- c/RConn1
  Current and Voltage Sensor (Three-Phase)/RConn4 -- b/RConn1
  Current and Voltage Sensor (Three-Phase)/RConn3 -- a/RConn1
  Current and Voltage Sensor (Three-Phase)/LConn3 -- C/RConn1
  Current and Voltage Sensor (Three-Phase)/LConn1 -- A/RConn1
  Current and Voltage Sensor (Three-Phase)/LConn2 -- B/RConn1

== system IEEE33_TR_TEMPORAL_RECOGNIZABILITY_MASTER/Bus_13/CB3-2 ==
  com : Inport
  Add : Sum
  Circuit Breaker : ee_lib/Switches & Breakers/Circuit Breaker (Three-Phase)  port_option=ee.enum.threePhasePort.expanded  control_port_option=ee.enum.controlport.ps  R_closed=0.01 Ohm  G_open=Three_PhaseBreaker_class('open',1000000,Inf,[0.0166666666666667 0.0833333333333333],'on').objParamMappingDerived.NewDerivedParam.G_open 1/Ohm  threshold=0.5 V  breaker_behavior=ee.enum.switches.breakerBehavior.zeroCrossingEnable  i_th=1e-8 A
  Data Type Conversion : DataTypeConversion  OutDataTypeStr=double  SaturateOnIntegerOverflow=off  RndMeth=Floor
  NOT : Logic  Operator=NOT  IconShape=distinctive  AllPortsSameDT=off  OutDataTypeStr=boolean
  Simulink-PS Converter : nesl_utility/Simulink-PS Converter  PhysicalDomain=network_engine_domain  SubClassName=ps_input  LeftPortType=input  RightPortType=output  PseudoPeriodic=off  Frequencies=[]  NoiseDistribution=none  NoiseParameters=[]  Unit=1  AffineConversion=off  FilteringAndDerivatives=provide  SimscapeFilterOrder=1  InputFilterTimeConstant=0.001  UdotUserProvided=0
  Step : Step  Time=1e-6  InitialValue=Three_PhaseBreaker_class('open',1000000,Inf,[0.0166666666666667 0.0833333333333333],'on').objParamMappingDerived.NewDerivedParam.StepInitialValue  FinalValue=0  SampleTime=0
  A : PMIOPort  Side=Left
  B : PMIOPort  Port=2  Side=Left
  C : PMIOPort  Port=3  Side=Left
  a : PMIOPort  Port=4  Side=Right
  b : PMIOPort  Port=5  Side=Right
  c : PMIOPort  Port=6  Side=Right
  wires:
  com/1 -> Add/1
  Add/1 -> NOT/1
  Step/1 -> Add/2
  Data Type Conversion/1 -> Simulink-PS Converter/1
  NOT/1 -> Data Type Conversion/1
  connections:
  Circuit Breaker/LConn1 -- Simulink-PS Converter/RConn1
  c/RConn1 -- Circuit Breaker/RConn3
  b/RConn1 -- Circuit Breaker/RConn2
  a/RConn1 -- Circuit Breaker/RConn1
  Circuit Breaker/LConn4 -- C/RConn1
  Circuit Breaker/LConn3 -- B/RConn1
  Circuit Breaker/LConn2 -- A/RConn1

== system IEEE33_TR_TEMPORAL_RECOGNIZABILITY_MASTER/Bus_13/VI Recorder16 ==
  Vrec : Inport
  Irec : Inport  Port=2
  tag scope: I12to13=global, V12to13=global
  wires:
  Vrec/1 -> [V12to13]
  Irec/1 -> [I12to13]

== system IEEE33_TR_TEMPORAL_RECOGNIZABILITY_MASTER/Bus_14/Bus Load 14 ==
  Electrical Reference : fl_lib/Electrical/Electrical Elements/Electrical Reference
  Wye-Connected Load : ee_lib/Passive/RLC Assemblies/Wye-Connected Load  port_option=ee.enum.threePhasePort.expanded  parameterization=2  component_structure=4  component_structure_PQ=4  R=1 Ohm  L=0.001 H  C=1e-6 F  VRated=11629.7798 V  FRated=60 Hz  P=120000 W  Qpos=80000 V*A  Qneg=Three_PhaseSeriesRLCLoad_class(0).objParamMappingDerived.NewDerivedParam.Qneg V*A  R_parasitic=1e-6 Ohm  G_parasitic=1e-6 1/Ohm  R_parasitic_PQ=1e-6 Ohm  G_parasitic_PQ=1e-6 1/Ohm  Vmag0=11629.7798 V  Vang0=0 deg  Freq0=60 Hz  IL_specify=on  IL_priority=High  IL=[ 0 0 0 ] A  IL_nominal_specify=off  IL_nominal_value=1  IL_nominal_unit=A  VC_specify=on  VC_priority=High  VC=[ 0 0 0 ] V  VC_nominal_specify=off  VC_nominal_value=1  VC_nominal_unit=V
  A : PMIOPort  Side=Left
  B : PMIOPort  Port=2  Side=Left
  C : PMIOPort  Port=3  Side=Left
  connections:
  Electrical Reference/LConn1 -- Wye-Connected Load/RConn1
  Wye-Connected Load/LConn3 -- C/RConn1
  Wye-Connected Load/LConn1 -- A/RConn1
  Wye-Connected Load/LConn2 -- B/RConn1

== system IEEE33_TR_TEMPORAL_RECOGNIZABILITY_MASTER/Bus_14/Bus_14 ==
  Current and Voltage Sensor (Three-Phase) : ee_lib/Sensors & Transducers/Current and Voltage Sensor (Three-Phase)  port_option=ee.enum.threePhasePort.expanded  vMeasurementType=1  outputUnit=2  SRated=100000000 V*A  VRated=500000 V  I_specify=off  I_priority=None  I=[ 0 0 0 ] A  I_nominal_specify=off  I_nominal_value=1  I_nominal_unit=A  V_specify=off  V_priority=None  V=[ 0 0 0 ] V  V_nominal_specify=off  V_nominal_value=1  V_nominal_unit=V
  Igain : Gain  Gain=Three_PhaseV_IMeasuremen_class('phase-to-phase','yes','off','off','off',100000000,500000).objParamMappingDerived.NewDerivedParam.IG
  PS-Simulink Converter : nesl_utility/PS-Simulink Converter  PhysicalDomain=network_engine_domain  SubClassName=ps_output  LeftPortType=input  RightPortType=output  PseudoPeriodic=off  Frequencies=[]  VectorFormat=1-D array  Unit=1  AffineConversion=off
  PS-Simulink Converter1 : nesl_utility/PS-Simulink Converter  PhysicalDomain=network_engine_domain  SubClassName=ps_output  LeftPortType=input  RightPortType=output  PseudoPeriodic=off  Frequencies=[]  VectorFormat=1-D array  Unit=1  AffineConversion=off
  Vgain : Gain  Gain=Three_PhaseV_IMeasuremen_class('phase-to-phase','yes','off','off','off',100000000,500000).objParamMappingDerived.NewDerivedParam.VG
  A : PMIOPort  Side=Left
  B : PMIOPort  Port=2  Side=Left
  C : PMIOPort  Port=3  Side=Left
  a : PMIOPort  Port=4  Side=Right
  b : PMIOPort  Port=5  Side=Right
  c : PMIOPort  Port=6  Side=Right
  Vabc : Outport  VectorParamsAs1DForOutWhenUnconnected=off
  Iabc : Outport  Port=2  VectorParamsAs1DForOutWhenUnconnected=off
  wires:
  Igain/1 -> Iabc/1
  Vgain/1 -> Vabc/1
  PS-Simulink Converter1/1 -> Igain/1
  PS-Simulink Converter/1 -> Vgain/1
  connections:
  Current and Voltage Sensor (Three-Phase)/RConn1 -- PS-Simulink Converter/LConn1
  Current and Voltage Sensor (Three-Phase)/RConn2 -- PS-Simulink Converter1/LConn1
  Current and Voltage Sensor (Three-Phase)/RConn5 -- c/RConn1
  Current and Voltage Sensor (Three-Phase)/RConn4 -- b/RConn1
  Current and Voltage Sensor (Three-Phase)/RConn3 -- a/RConn1
  Current and Voltage Sensor (Three-Phase)/LConn3 -- C/RConn1
  Current and Voltage Sensor (Three-Phase)/LConn1 -- A/RConn1
  Current and Voltage Sensor (Three-Phase)/LConn2 -- B/RConn1

== system IEEE33_TR_TEMPORAL_RECOGNIZABILITY_MASTER/Bus_14/CB3-2 ==
  com : Inport
  Add : Sum
  Circuit Breaker : ee_lib/Switches & Breakers/Circuit Breaker (Three-Phase)  port_option=ee.enum.threePhasePort.expanded  control_port_option=ee.enum.controlport.ps  R_closed=0.01 Ohm  G_open=Three_PhaseBreaker_class('open',1000000,Inf,[0.0166666666666667 0.0833333333333333],'on').objParamMappingDerived.NewDerivedParam.G_open 1/Ohm  threshold=0.5 V  breaker_behavior=ee.enum.switches.breakerBehavior.zeroCrossingEnable  i_th=1e-8 A
  Data Type Conversion : DataTypeConversion  OutDataTypeStr=double  SaturateOnIntegerOverflow=off  RndMeth=Floor
  NOT : Logic  Operator=NOT  IconShape=distinctive  AllPortsSameDT=off  OutDataTypeStr=boolean
  Simulink-PS Converter : nesl_utility/Simulink-PS Converter  PhysicalDomain=network_engine_domain  SubClassName=ps_input  LeftPortType=input  RightPortType=output  PseudoPeriodic=off  Frequencies=[]  NoiseDistribution=none  NoiseParameters=[]  Unit=1  AffineConversion=off  FilteringAndDerivatives=provide  SimscapeFilterOrder=1  InputFilterTimeConstant=0.001  UdotUserProvided=0
  Step : Step  Time=1e-6  InitialValue=Three_PhaseBreaker_class('open',1000000,Inf,[0.0166666666666667 0.0833333333333333],'on').objParamMappingDerived.NewDerivedParam.StepInitialValue  FinalValue=0  SampleTime=0
  A : PMIOPort  Side=Left
  B : PMIOPort  Port=2  Side=Left
  C : PMIOPort  Port=3  Side=Left
  a : PMIOPort  Port=4  Side=Right
  b : PMIOPort  Port=5  Side=Right
  c : PMIOPort  Port=6  Side=Right
  wires:
  com/1 -> Add/1
  Add/1 -> NOT/1
  Step/1 -> Add/2
  Data Type Conversion/1 -> Simulink-PS Converter/1
  NOT/1 -> Data Type Conversion/1
  connections:
  Circuit Breaker/LConn1 -- Simulink-PS Converter/RConn1
  c/RConn1 -- Circuit Breaker/RConn3
  b/RConn1 -- Circuit Breaker/RConn2
  a/RConn1 -- Circuit Breaker/RConn1
  Circuit Breaker/LConn4 -- C/RConn1
  Circuit Breaker/LConn3 -- B/RConn1
  Circuit Breaker/LConn2 -- A/RConn1

== system IEEE33_TR_TEMPORAL_RECOGNIZABILITY_MASTER/Bus_14/VI Recorder17 ==
  Vrec : Inport
  Irec : Inport  Port=2
  tag scope: I13to14=global, V13to14=global
  wires:
  Vrec/1 -> [V13to14]
  Irec/1 -> [I13to14]

== system IEEE33_TR_TEMPORAL_RECOGNIZABILITY_MASTER/Bus_15/Bus Load 15 ==
  Electrical Reference : fl_lib/Electrical/Electrical Elements/Electrical Reference
  Wye-Connected Load : ee_lib/Passive/RLC Assemblies/Wye-Connected Load  port_option=ee.enum.threePhasePort.expanded  parameterization=2  component_structure=4  component_structure_PQ=4  R=1 Ohm  L=0.001 H  C=1e-6 F  VRated=11611.9419 V  FRated=60 Hz  P=60000 W  Qpos=10000 V*A  Qneg=Three_PhaseSeriesRLCLoad_class(0).objParamMappingDerived.NewDerivedParam.Qneg V*A  R_parasitic=1e-6 Ohm  G_parasitic=1e-6 1/Ohm  R_parasitic_PQ=1e-6 Ohm  G_parasitic_PQ=1e-6 1/Ohm  Vmag0=11611.9419 V  Vang0=0 deg  Freq0=60 Hz  IL_specify=on  IL_priority=High  IL=[ 0 0 0 ] A  IL_nominal_specify=off  IL_nominal_value=1  IL_nominal_unit=A  VC_specify=on  VC_priority=High  VC=[ 0 0 0 ] V  VC_nominal_specify=off  VC_nominal_value=1  VC_nominal_unit=V
  A : PMIOPort  Side=Left
  B : PMIOPort  Port=2  Side=Left
  C : PMIOPort  Port=3  Side=Left
  connections:
  Electrical Reference/LConn1 -- Wye-Connected Load/RConn1
  Wye-Connected Load/LConn3 -- C/RConn1
  Wye-Connected Load/LConn1 -- A/RConn1
  Wye-Connected Load/LConn2 -- B/RConn1
